simulink model "testLPVOL"  (R2019b)
settings: Solver=VariableStepAuto  StartTime=0.0  StopTime=10.0  RelTol=1e-3
values from neighbouring files (symbols this model uses):
  OutList = OutTable.Properties.VariableNames    [initLPVParam.m]    (also in testCtrl.m; testOutList.m = cell(40, 1); testqLPV.m = cell(40, 1))
undefined symbols (not defined in the file or in its folder): strmatch, sys12d_w
libraries: cstblocks x1
settings Model: Creator=ditt_aj  LastModifiedBy=ditt_aj

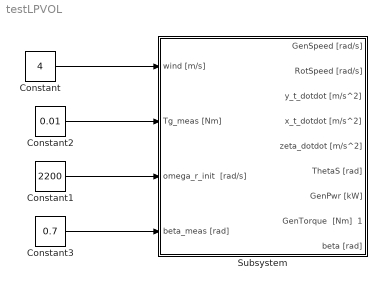
== system testLPVOL ==
  Constant : Constant  Value=4
  Constant1 : Constant  Value=2200
  Constant2 : Constant  Value=0.01
  Constant3 : Constant  Value=0.7
  Subsystem : Subsystem
  wires:
  Constant/1 -> Subsystem/1(wind [m/s])
  Constant2/1 -> Subsystem/2(Tg_meas [Nm])
  Constant3/1 -> Subsystem/4(beta_meas [rad])
  Constant1/1 -> Subsystem/3(omega_r_init  [rad/s])

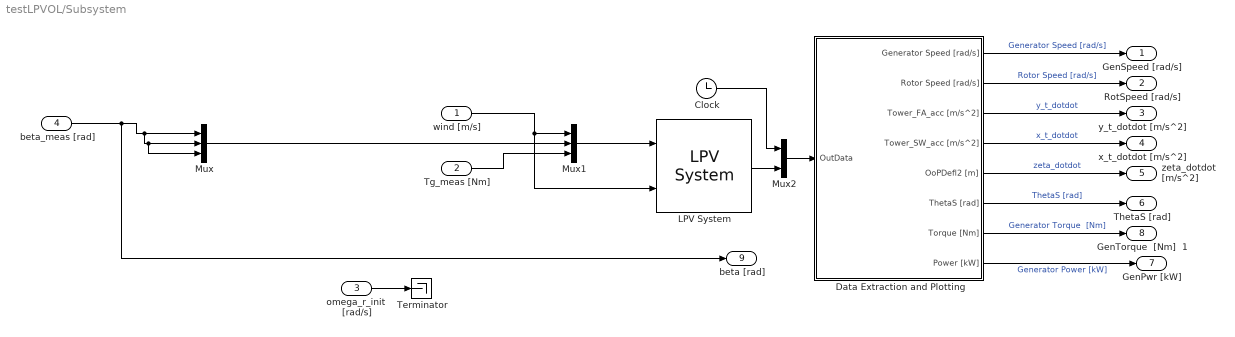
== system testLPVOL/Subsystem ==
  wind [m/s] : Inport
  Tg_meas [Nm] : Inport  Port=2
  omega_r_init  [rad/s] : Inport  Port=3
  beta_meas [rad] : Inport  Port=4
  Clock : Clock
  Data Extraction and Plotting : Subsystem
  LPV System : cstblocks/Linear Parameter Varying/LPV System  sys=sysd  x0=x0  uOffset=uoff  yOffset=yoff  xOffset=xoff  opEquilOption=on  dxOffset=0  sysFixedOption=Use the first model in state-space array  sysFixed=sys12d_w(:,:,4)  AFixed=false  BFixed=false  CFixed=false  DFixed=false  uDelayFixed=false  yDelayFixed=false  iDelayFixed=false  IMethod=Nearest  EMethod=Clip  IndexSearch=Binary search  IndexBegin=on  OutputX=off  OutputXdot=off  OutputLTI=off  OutputOP=off  DataType=double  SimMode=Interpreted execution  InitBufferSize=1024  FixedBuffer=off
      settings: SourceProductName=Control System Toolbox  SourceProductBaseCode=CT
  Mux : Mux  Inputs=3
  Mux1 : Mux  Inputs=3
  Mux2 : Mux  Inputs=2
  Terminator : Terminator
  "GenSpeed [rad/s] " : Outport  VectorParamsAs1DForOutWhenUnconnected=off
  " RotSpeed [rad/s]" : Outport  Port=2  VectorParamsAs1DForOutWhenUnconnected=off
  y_t_dotdot [m/s^2] : Outport  Port=3  VectorParamsAs1DForOutWhenUnconnected=off
  x_t_dotdot [m/s^2] : Outport  Port=4  VectorParamsAs1DForOutWhenUnconnected=off
  zeta_dotdot [m/s^2] : Outport  Port=5  VectorParamsAs1DForOutWhenUnconnected=off
  ThetaS [rad] : Outport  Port=6  VectorParamsAs1DForOutWhenUnconnected=off
  GenPwr [kW] : Outport  Port=7  VectorParamsAs1DForOutWhenUnconnected=off
  GenTorque  [Nm]  1 : Outport  Port=8  VectorParamsAs1DForOutWhenUnconnected=off
  beta [rad] : Outport  Port=9  VectorParamsAs1DForOutWhenUnconnected=off
  wires:
  beta_meas [rad]/1 -> beta [rad]/1, Mux/3, Mux/2, Mux/1
  Mux1/1 -> LPV System/1
  Data Extraction and Plotting/5(OoPDefl2 [m]) -> zeta_dotdot [m/s^2]/1  "zeta_dotdot"
  Data Extraction and Plotting/6(ThetaS [rad]) -> ThetaS [rad]/1  "ThetaS [rad]"
  Data Extraction and Plotting/2(Rotor Speed [rad/s]) -> " RotSpeed [rad/s]"/1  "Rotor Speed [rad/s]"
  Data Extraction and Plotting/8(Power [kW]) -> GenPwr [kW]/1  "Generator Power [kW]"
  omega_r_init  [rad/s]/1 -> Terminator/1
  Mux/1 -> Mux1/2
  Data Extraction and Plotting/1(Generator Speed [rad/s]) -> "GenSpeed [rad/s] "/1  "Generator Speed [rad/s]"
  Data Extraction and Plotting/7(Torque [Nm]) -> GenTorque  [Nm]  1/1  "Generator Torque  [Nm]"
  Data Extraction and Plotting/4(Tower_SW_acc [m/s^2]) -> x_t_dotdot [m/s^2]/1  "x_t_dotdot"
  Data Extraction and Plotting/3(Tower_FA_acc [m/s^2]) -> y_t_dotdot [m/s^2]/1  "y_t_dotdot"
  wind [m/s]/1 -> LPV System/2, Mux1/1
  Mux2/1 -> Data Extraction and Plotting/1(OutData)
  Tg_meas [Nm]/1 -> Mux1/3
  Clock/1 -> Mux2/1
  LPV System/1 -> Mux2/2

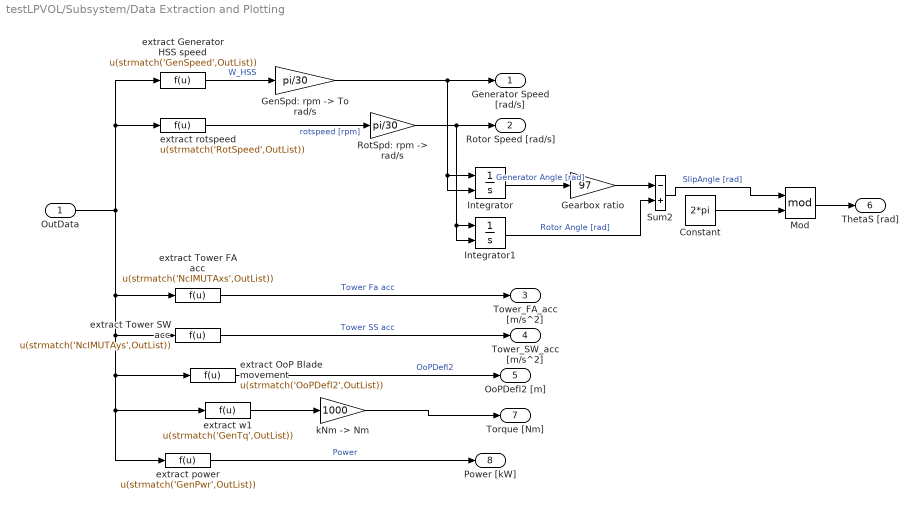
== system testLPVOL/Subsystem/Data Extraction and Plotting ==
  OutData : Inport
  Constant : Constant  Value=2*pi
  Gearbox ratio : Gain  Gain=97
  "GenSpd: rpm -> To rad/s" : Gain  Gain=pi/30
  Integrator : Integrator  InitialConditionSource=external
  Integrator1 : Integrator  InitialConditionSource=external
  Mod : Math  Operator=mod  SignedPower=off  SaturateOnIntegerOverflow=on
  "RotSpd: rpm -> rad/s" : Gain  Gain=pi/30
  Sum2 : Sum  Inputs=-+
  extract Generator HSS speed : Fcn  Expr=u(strmatch('GenSpeed',OutList))
  extract OoP Blade movement : Fcn  Expr=u(strmatch('OoPDefl2',OutList))
  extract Tower FA acc : Fcn  Expr=u(strmatch('NcIMUTAxs',OutList))
  extract Tower SW acc : Fcn  Expr=u(strmatch('NcIMUTAys',OutList))
  extract power : Fcn  Expr=u(strmatch('GenPwr',OutList))
  extract rotspeed : Fcn  Expr=u(strmatch('RotSpeed',OutList))
  extract w1 : Fcn  Expr=u(strmatch('GenTq',OutList))
  "kNm -> Nm" : Gain  Gain=1000
  Generator Speed [rad/s] : Outport  VectorParamsAs1DForOutWhenUnconnected=off
  Rotor Speed [rad/s] : Outport  Port=2  VectorParamsAs1DForOutWhenUnconnected=off
  Tower_FA_acc [m/s^2] : Outport  Port=3  VectorParamsAs1DForOutWhenUnconnected=off
  Tower_SW_acc [m/s^2] : Outport  Port=4  VectorParamsAs1DForOutWhenUnconnected=off
  OoPDefl2 [m] : Outport  Port=5  VectorParamsAs1DForOutWhenUnconnected=off
  ThetaS [rad] : Outport  Port=6  VectorParamsAs1DForOutWhenUnconnected=off
  Torque [Nm] : Outport  Port=7  VectorParamsAs1DForOutWhenUnconnected=off
  Power [kW] : Outport  Port=8  VectorParamsAs1DForOutWhenUnconnected=off
  wires:
  extract rotspeed/1 -> "RotSpd: rpm -> rad/s"/1  "rotspeed [rpm]"
  extract power/1 -> Power [kW]/1  "Power"
  extract Tower FA acc/1 -> Tower_FA_acc [m/s^2]/1  "Tower Fa acc"
  extract Tower SW acc/1 -> Tower_SW_acc [m/s^2]/1  "Tower SS acc"
  extract w1/1 -> "kNm -> Nm"/1
  "kNm -> Nm"/1 -> Torque [Nm]/1
  "RotSpd: rpm -> rad/s"/1 -> Integrator1/2, Integrator1/1, Rotor Speed [rad/s]/1
  "GenSpd: rpm -> To rad/s"/1 -> Integrator/2, Integrator/1, Generator Speed [rad/s]/1
  extract Generator HSS speed/1 -> "GenSpd: rpm -> To rad/s"/1  "W_HSS"
  extract OoP Blade movement/1 -> OoPDefl2 [m]/1  "OoPDefl2"
  OutData/1 -> extract power/1, extract w1/1, extract OoP Blade movement/1, extract Tower SW acc/1, extract Tower FA acc/1, extract Generator HSS speed/1, extract rotspeed/1
  Integrator/1 -> Gearbox ratio/1  "Generator Angle [rad]"
  Integrator1/1 -> Sum2/2  "Rotor Angle [rad]"
  Sum2/1 -> Mod/1  "SlipAngle [rad]"
  Constant/1 -> Mod/2
  Mod/1 -> ThetaS [rad]/1
  Gearbox ratio/1 -> Sum2/1
